simulink model "fi_sc"  (R2026a)
settings: Solver=VariableStepAuto  StopTime=40  FixedStep=0.1  MaxStep=.1
model workspace (MAT data in the model file):
  T = [0 0.05 0.1 0.15 0.2 0.25 0.3 0.35 0.4 0.45 0.5 0.55 ... (701 elements, 701x1)]
  U = [3.99594136536 3.99594136536 3.99594136536 3.99594136536 3.99594136536 3.99594136536 3.99594136536 3.99594136536 3.99594136536 3.99594136536 3.99594136536 3.99594136536 ... (701 elements, 701x1)]
libraries: neural x11, simulink_extras x2
settings Model: Creator=syaghoub  LastModifiedBy=harry_31916
settings DataIOCC: ExternalInput=simin

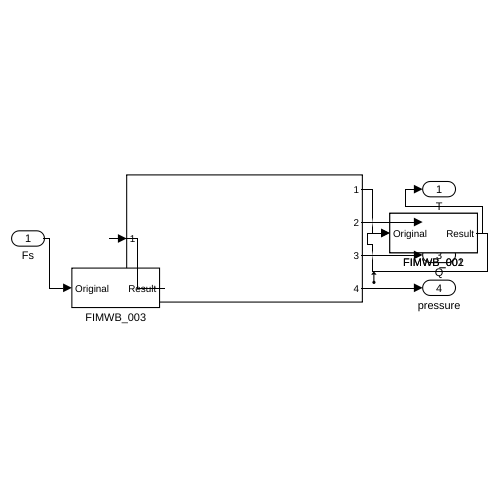
[thumbnail: Simulink's stored preview of the top-level diagram]
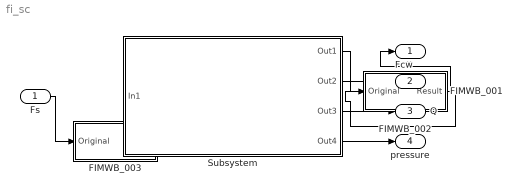
== system fi_sc ==
  Fs : Inport
  FIMWB_001 : Subsystem  Tag=fimwb.fault.1
  FIMWB_002 : Subsystem  Tag=fimwb.fault.2
  FIMWB_003 : Subsystem  Tag=fimwb.fault.3
  Subsystem : Subsystem
  T : Outport  VectorParamsAs1DForOutWhenUnconnected=off
  Fcw : Outport  Port=2  VectorParamsAs1DForOutWhenUnconnected=off
  Q : Outport  Port=3  VectorParamsAs1DForOutWhenUnconnected=off
  pressure : Outport  Port=4  VectorParamsAs1DForOutWhenUnconnected=off
  wires:
  Subsystem/2(Out2) -> Fcw/1
  Subsystem/3(Out3) -> Q/1
  Subsystem/4(Out4) -> pressure/1
  Subsystem/1(Out1) -> FIMWB_001/1(Original)
  FIMWB_001/1(Result) -> FIMWB_002/1(Original)
  FIMWB_002/1(Result) -> T/1
  Fs/1 -> FIMWB_003/1(Original)
  FIMWB_003/1(Result) -> Subsystem/1(In1)

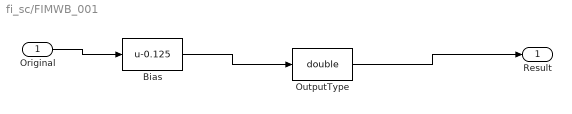
== system fi_sc/FIMWB_001 ==
  Original : Inport
  Bias : Bias  Bias=-0.125  SaturateOnIntegerOverflow=off
  OutputType : DataTypeConversion  OutDataTypeStr=double  RndMeth=Round
  Result : Outport
  wires:
  Original/1 -> Bias/1
  Bias/1 -> OutputType/1
  OutputType/1 -> Result/1

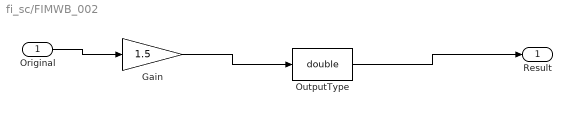
== system fi_sc/FIMWB_002 ==
  Original : Inport
  Gain : Gain  Gain=1.5  OutDataTypeStr=Inherit: Same as input
  OutputType : DataTypeConversion  OutDataTypeStr=double  RndMeth=Round
  Result : Outport
  wires:
  Original/1 -> Gain/1
  Gain/1 -> OutputType/1
  OutputType/1 -> Result/1

== system fi_sc/FIMWB_003 ==
  Original : Inport
  Bias : Bias  Bias=0.015625  SaturateOnIntegerOverflow=off
  OutputType : DataTypeConversion  OutDataTypeStr=double  RndMeth=Round
  Result : Outport
  wires:
  Original/1 -> Bias/1
  Bias/1 -> OutputType/1
  OutputType/1 -> Result/1

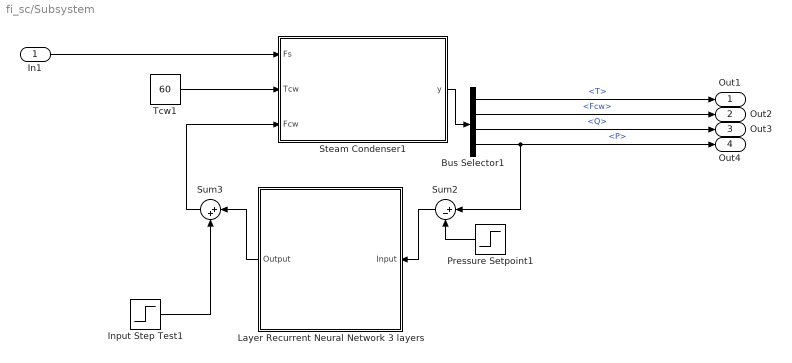
== system fi_sc/Subsystem ==
  In1 : Inport
  Bus Selector1 : BusSelector  OutputSignals=T,Fcw,Q,P
  Input Step Test1 : Step  Time=10  FinalValue=0  SampleTime=0
  "Layer Recurrent Neural Network 3 layers " : Subsystem  mask{ai_layer_1_delayed_1=[0;0;0], ai_layer_1_delayed_2=[0;0;0], Parameter3=[]}
      mask prompts: ai_layer_1_delayed_1 "Initial layer 1 state at timestep 0."; ai_layer_1_delayed_2 "Initial layer 1 state at timestep -1."
      mask help: Layer Recurrent Neural Network
      mask Display: e = 0.06;c1 = [120 150 230]/255;c2 = ([120 150 230]+0)/383;c3 = ([120 150 230]+128)/383;patch([0 1 1 0],[0 0 1 1],c1);patch([0 1 1 1-e 1-e 0+e],[0 0 1 1-e 0+e 0+e],c2);patch([0 0 1 1-e 0+e 0+e],[0 1 1 1-e 1-e 0+e],c3);plot([0 1 1 0 0],[0 0 1 1 0]);fprintf('NNET');port_label('input',1,' Input');port_label('output',1,'Output ');
  Pressure Setpoint1 : Step  Time=2  InitialValue=90  FinalValue=87  SampleTime=0
  Steam Condenser1 : Subsystem  mask{V=3, Mcw=500, UA=356.972413581334, tau=1, Fcw=107.8880952381, P=90, T=80}
      mask prompts: V "Volume [m3]"; Mcw "CW Holdup [kg]"; UA "UA [kW/K]"; tau "Actuator time constant [s]"; Fcw "Fcw [kg/s]"; P "P [kPa]"; T "T [degC]"
      mask init:
      | y1=[.3 .3 .7 .7 .3 NaN .4 .4 NaN .5 .5 NaN .6 .6 NaN 0.2 0.3 NaN 0.7 0.8 NaN 0.7 0.8 NaN 0.82 NaN 0.18];
      | x1=[.8 .2 .2 .8 .8 NaN .8 .2 NaN .8 .2 NaN .8 .2 NaN 0.5 0.5 NaN 0.3 0.3 NaN 0.7 0.7 NaN -0.05 NaN 1.05];
      | y2=0.3:0.05:0.7;
      | x2=sqrt(0.0625-(y2-0.5).^2);
      | y3=[.5 .5 .8 NaN 0.2 0.4 0.4];
      | x3=[x2(5)+0.65 0.95 0.95 NaN .1 .1 0.35-x2(3)];
      mask Display:
      | plot([x1 NaN 0.65+x2 NaN 0.35-x2 NaN x3],[y1 NaN y2 NaN y2 NaN y3])
      | port_label('input',1,'Fs')
      | port_label('input',2,'Tcw')
      | port_label('input',3,'Fcw')
      | port_label('output',1,'y')
  Sum2 : Sum  Inputs=|+-  InputSameDT=on  OutDataTypeStr=Inherit: Same as first input
  Sum3 : Sum  Inputs=|++  InputSameDT=on  OutDataTypeStr=Inherit: Same as first input
  Tcw1 : Constant  Value=60  VectorParams1D=off
  Out1 : Outport  VectorParamsAs1DForOutWhenUnconnected=off
  Out2 : Outport  Port=2  VectorParamsAs1DForOutWhenUnconnected=off
  Out3 : Outport  Port=3  VectorParamsAs1DForOutWhenUnconnected=off
  Out4 : Outport  Port=4  VectorParamsAs1DForOutWhenUnconnected=off
  wires:
  Bus Selector1/4 -> Out4/1, Sum2/1  "<P>"
  Bus Selector1/3 -> Out3/1  "<Q>"
  Tcw1/1 -> Steam Condenser1/2(Tcw)
  Sum3/1 -> Steam Condenser1/3(Fcw)
  Bus Selector1/1 -> Out1/1  "<T>"
  Steam Condenser1/1(y) -> Bus Selector1/1
  Bus Selector1/2 -> Out2/1  "<Fcw>"
  Pressure Setpoint1/1 -> Sum2/2
  Input Step Test1/1 -> Sum3/2
  In1/1 -> Steam Condenser1/1(Fs)
  Sum2/1 -> "Layer Recurrent Neural Network 3 layers "/1(Input)
  "Layer Recurrent Neural Network 3 layers "/1(Output) -> Sum3/1

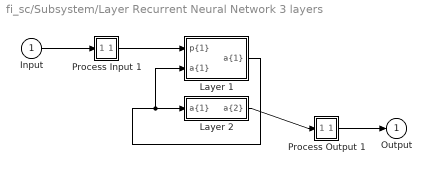
== system fi_sc/Subsystem/Layer Recurrent Neural Network 3 layers  ==
  Input : Inport  PortDimensions=1
      mask Display: e = 0.06;c1 = [120 230 180]/255;c2 = ([120 230 180]+0)/(256+128);c3 = ([120 230 180]+128)/(256+128);patch([0 1 1 0],[0 0 1 1],c1);patch([0 1 1 1-e 1-e 0+e],[0 0 1 1-e 0+e 0+e],c2);patch([0 0 1 1-e 0+e 0+e],[0 1 1 1-e 1-e 0+e],c3);plot([0 1 1 0 0],[0 0 1 1 0]);
  Layer 1 : Subsystem
      mask Display: e = 0.06;c1 = [120 150 230]/255;c2 = ([120 150 230]+0)/383;c3 = ([120 150 230]+128)/383;patch([0 1 1 0],[0 0 1 1],c1);patch([0 1 1 1-e 1-e 0+e],[0 0 1 1-e 0+e 0+e],c2);patch([0 0 1 1-e 0+e 0+e],[0 1 1 1-e 1-e 0+e],c3);plot([0 1 1 0 0],[0 0 1 1 0]);
  Layer 2 : Subsystem
      mask Display: e = 0.06;c1 = [120 150 230]/255;c2 = ([120 150 230]+0)/383;c3 = ([120 150 230]+128)/383;patch([0 1 1 0],[0 0 1 1],c1);patch([0 1 1 1-e 1-e 0+e],[0 0 1 1-e 0+e 0+e],c2);patch([0 0 1 1-e 0+e 0+e],[0 1 1 1-e 1-e 0+e],c3);plot([0 1 1 0 0],[0 0 1 1 0]);
  Process Input 1 : Subsystem
      mask Display: e = 0.06;c1 = [120 150 230]/255;c2 = ([120 150 230]+0)/383;c3 = ([120 150 230]+128)/383;patch([0 1 1 0],[0 0 1 1],c1);patch([0 1 1 1-e 1-e 0+e],[0 0 1 1-e 0+e 0+e],c2);patch([0 0 1 1-e 0+e 0+e],[0 1 1 1-e 1-e 0+e],c3);plot([0 1 1 0 0],[0 0 1 1 0]);
  Process Output 1 : Subsystem
      mask Display: e = 0.06;c1 = [120 150 230]/255;c2 = ([120 150 230]+0)/383;c3 = ([120 150 230]+128)/383;patch([0 1 1 0],[0 0 1 1],c1);patch([0 1 1 1-e 1-e 0+e],[0 0 1 1-e 0+e 0+e],c2);patch([0 0 1 1-e 0+e 0+e],[0 1 1 1-e 1-e 0+e],c3);plot([0 1 1 0 0],[0 0 1 1 0]);
  Output : Outport  InitialOutput=0  VectorParamsAs1DForOutWhenUnconnected=off
      mask Display: e = 0.06;c1 = [120 230 180]/255;c2 = ([120 230 180]+0)/(256+128);c3 = ([120 230 180]+128)/(256+128);patch([0 1 1 0],[0 0 1 1],c1);patch([0 1 1 1-e 1-e 0+e],[0 0 1 1-e 0+e 0+e],c2);patch([0 0 1 1-e 0+e 0+e],[0 1 1 1-e 1-e 0+e],c3);plot([0 1 1 0 0],[0 0 1 1 0]);
  wires:
  Layer 1/1("a{1}") -> Layer 1/2("a{1} "), Layer 2/1("a{1} ")
  Process Input 1/1(p) -> Layer 1/1("p{1}")
  Layer 2/1("a{2}") -> Process Output 1/1(a)
  Input/1 -> Process Input 1/1(x)
  Process Output 1/1(y) -> Output/1

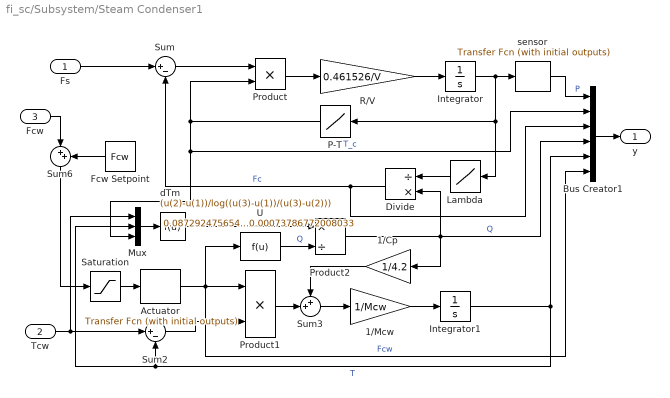
== system fi_sc/Subsystem/Steam Condenser1 ==
  Fs : Inport
  Tcw : Inport  Port=2
  Fcw : Inport  Port=3
  1/Cp : Gain  Gain=1/4.2  OutDataTypeStr=Inherit: Same as input  ParamDataTypeStr=Inherit: Same as input
  1/Mcw : Gain  Gain=1/Mcw  OutDataTypeStr=Inherit: Same as input  ParamDataTypeStr=Inherit: Same as input
  Actuator : simulink_extras/Additional Linear/Transfer Fcn (with initial outputs)  N=[1]  D=[tau 1]  Y0=Fcw  U0=Fcw
  Bus Creator1 : BusCreator  Inputs=6
  Divide : Product  Inputs=/*  InputSameDT=on  RndMeth=Zero  OutDataTypeStr=Inherit: Same as first input
  Fcw Setpoint : Constant  Value=Fcw
  Integrator : Integrator  InitialCondition=P
  Integrator1 : Integrator  InitialCondition=T
  Lambda : Lookup  InputValues=[50 60 70 80 90 100 110]  Table=[2305.42 2293.64 2283.30 2274.05 2265.65 2257.92 2250.76]
  Mux : Mux  Inputs=3
  P-T : Lookup  InputValues=[50 60 70 80 90 100 110]  Table=[81.3167 85.9258 89.9315 93.4854 96.6870 99.6059 102.2923]
  Product : Product  InputSameDT=on  RndMeth=Zero  OutDataTypeStr=Inherit: Same as first input
  Product1 : Product  InputSameDT=on  RndMeth=Zero  OutDataTypeStr=Inherit: Same as first input
  Product2 : Product  Inputs=*/  InputSameDT=on  RndMeth=Zero  OutDataTypeStr=Inherit: Same as first input
  R/V : Gain  Gain=0.461526/V  OutDataTypeStr=Inherit: Same as input  ParamDataTypeStr=Inherit: Same as input
  Saturation : Saturate  UpperLimit=200  LowerLimit=0
  Sum : Sum  Inputs=|+-  InputSameDT=on  OutDataTypeStr=Inherit: Same as first input
  Sum2 : Sum  Inputs=|+-  InputSameDT=on  OutDataTypeStr=Inherit: Same as first input
  Sum3 : Sum  Inputs=++|  InputSameDT=on  OutDataTypeStr=Inherit: Same as first input
  Sum6 : Sum  Inputs=|++  InputSameDT=on  OutDataTypeStr=Inherit: Same as first input
  U : Fcn  Expr=0.0872924756541668/u^0.8+0.00073786772008033
  dTm : Fcn  Expr=(u(2)-u(1))/log((u(3)-u(1))/(u(3)-u(2)))
  sensor : simulink_extras/Additional Linear/Transfer Fcn (with initial outputs)  N=[1]  D=[tau/2 1]  Y0=P  U0=P
  y : Outport  VectorParamsAs1DForOutWhenUnconnected=off
  wires:
  R/V/1 -> Integrator/1
  Product/1 -> R/V/1
  Sum/1 -> Product/1
  Fs/1 -> Sum/1
  Integrator/1 -> sensor/1, Lambda/1, P-T/1
  1/Mcw/1 -> Integrator1/1
  Integrator1/1 -> Sum2/2, Mux/2, Bus Creator1/5  "T"
  Tcw/1 -> Sum2/1, Mux/1
  Sum2/1 -> Product1/2
  Product1/1 -> Sum3/2
  Sum3/1 -> 1/Mcw/1
  1/Cp/1 -> Sum3/1
  dTm/1 -> Product2/1
  Bus Creator1/1 -> y/1
  Actuator/1 -> Product1/1, U/1, Bus Creator1/6  "Fcw"
  sensor/1 -> Bus Creator1/1  "P"
  Saturation/1 -> Actuator/1
  Sum6/1 -> Saturation/1
  Fcw/1 -> Sum6/1
  Fcw Setpoint/1 -> Sum6/2
  Lambda/1 -> Divide/1
  Divide/1 -> Sum/2, Bus Creator1/3  "Fc"
  P-T/1 -> Product/2, Mux/3, Bus Creator1/2  "T_c"
  Mux/1 -> dTm/1
  Product2/1 -> 1/Cp/1, Divide/2, Bus Creator1/4  "Q"
  U/1 -> Product2/2  "Q"

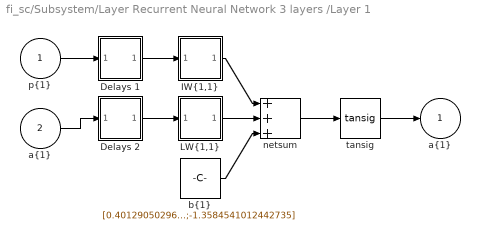
== system fi_sc/Subsystem/Layer Recurrent Neural Network 3 layers /Layer 1 ==
  "p{1}" : Inport  PortDimensions=1
      mask Display: e = 0.06;c1 = [120 230 180]/255;c2 = ([120 230 180]+0)/(256+128);c3 = ([120 230 180]+128)/(256+128);patch([0 1 1 0],[0 0 1 1],c1);patch([0 1 1 1-e 1-e 0+e],[0 0 1 1-e 0+e 0+e],c2);patch([0 0 1 1-e 0+e 0+e],[0 1 1 1-e 1-e 0+e],c3);plot([0 1 1 0 0],[0 0 1 1 0]);
  "a{1} " : Inport  Port=2  PortDimensions=3
      mask Display: e = 0.06;c1 = [120 230 180]/255;c2 = ([120 230 180]+0)/(256+128);c3 = ([120 230 180]+128)/(256+128);patch([0 1 1 0],[0 0 1 1],c1);patch([0 1 1 1-e 1-e 0+e],[0 0 1 1-e 0+e 0+e],c2);patch([0 0 1 1-e 0+e 0+e],[0 1 1 1-e 1-e 0+e],c3);plot([0 1 1 0 0],[0 0 1 1 0]);
  Delays 1 : Subsystem
      mask Display: e = 0.06;c1 = [120 150 230]/255;c2 = ([120 150 230]+0)/383;c3 = ([120 150 230]+128)/383;patch([0 1 1 0],[0 0 1 1],c1);patch([0 1 1 1-e 1-e 0+e],[0 0 1 1-e 0+e 0+e],c2);patch([0 0 1 1-e 0+e 0+e],[0 1 1 1-e 1-e 0+e],c3);plot([0 1 1 0 0],[0 0 1 1 0]);disp('0');
  Delays 2 : Subsystem
      mask Display: e = 0.06;c1 = [120 150 230]/255;c2 = ([120 150 230]+0)/383;c3 = ([120 150 230]+128)/383;patch([0 1 1 0],[0 0 1 1],c1);patch([0 1 1 1-e 1-e 0+e],[0 0 1 1-e 0+e 0+e],c2);patch([0 0 1 1-e 0+e 0+e],[0 1 1 1-e 1-e 0+e],c3);plot([0 1 1 0 0],[0 0 1 1 0]);disp('1-2');
  "IW{1,1}" : Subsystem
      mask Display: e = 0.06;c1 = [120 150 230]/255;c2 = ([120 150 230]+0)/383;c3 = ([120 150 230]+128)/383;patch([0 1 1 0],[0 0 1 1],c1);patch([0 1 1 1-e 1-e 0+e],[0 0 1 1-e 0+e 0+e],c2);patch([0 0 1 1-e 0+e 0+e],[0 1 1 1-e 1-e 0+e],c3);plot([0 1 1 0 0],[0 0 1 1 0]);disp('W');
  "LW{1,1}" : Subsystem
      mask Display: e = 0.06;c1 = [120 150 230]/255;c2 = ([120 150 230]+0)/383;c3 = ([120 150 230]+128)/383;patch([0 1 1 0],[0 0 1 1],c1);patch([0 1 1 1-e 1-e 0+e],[0 0 1 1-e 0+e 0+e],c2);patch([0 0 1 1-e 0+e 0+e],[0 1 1 1-e 1-e 0+e],c3);plot([0 1 1 0 0],[0 0 1 1 0]);disp('W');
  "b{1}" : Constant  Value=[0.40129050296348601;-0.12475735064274925;-1.3584541012442735]
      mask Display: e = 0.06;c1 = [120 150 230]/255;c2 = ([120 150 230]+0)/383;c3 = ([120 150 230]+128)/383;patch([0 1 1 0],[0 0 1 1],c1);patch([0 1 1 1-e 1-e 0+e],[0 0 1 1-e 0+e 0+e],c2);patch([0 0 1 1-e 0+e 0+e],[0 1 1 1-e 1-e 0+e],c3);plot([0 1 1 0 0],[0 0 1 1 0]);disp('b');
  netsum : Sum  Inputs=3  InputSameDT=on  SaturateOnIntegerOverflow=on  OutDataTypeStr=Inherit: Same as first input
      mask Display: e = 0.06;c1 = [120 150 230]/255;c2 = ([120 150 230]+0)/383;c3 = ([120 150 230]+128)/383;patch([0 1 1 0],[0 0 1 1],c1);patch([0 1 1 1-e 1-e 0+e],[0 0 1 1-e 0+e 0+e],c2);patch([0 0 1 1-e 0+e 0+e],[0 1 1 1-e 1-e 0+e],c3);plot([0 1 1 0 0],[0 0 1 1 0]);disp('+');
  tansig : neural/Transfer Functions/tansig
  "a{1}" : Outport  InitialOutput=[0;0;0]  VectorParamsAs1DForOutWhenUnconnected=off
      mask Display: e = 0.06;c1 = [120 230 180]/255;c2 = ([120 230 180]+0)/(256+128);c3 = ([120 230 180]+128)/(256+128);patch([0 1 1 0],[0 0 1 1],c1);patch([0 1 1 1-e 1-e 0+e],[0 0 1 1-e 0+e 0+e],c2);patch([0 0 1 1-e 0+e 0+e],[0 1 1 1-e 1-e 0+e],c3);plot([0 1 1 0 0],[0 0 1 1 0]);
  wires:
  "p{1}"/1 -> Delays 1/1("p{1}")
  Delays 1/1("pd{1,1}") -> "IW{1,1}"/1("pd{1,1}")
  "IW{1,1}"/1("iz{1,1}") -> netsum/1
  "a{1} "/1 -> Delays 2/1("p{1}")
  Delays 2/1("pd{1,1}") -> "LW{1,1}"/1("ad{1,1}")
  "LW{1,1}"/1("lz{1,1}") -> netsum/2
  "b{1}"/1 -> netsum/3
  netsum/1 -> tansig/1
  tansig/1 -> "a{1}"/1

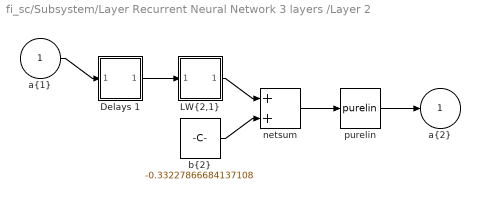
== system fi_sc/Subsystem/Layer Recurrent Neural Network 3 layers /Layer 2 ==
  "a{1} " : Inport  PortDimensions=3
      mask Display: e = 0.06;c1 = [120 230 180]/255;c2 = ([120 230 180]+0)/(256+128);c3 = ([120 230 180]+128)/(256+128);patch([0 1 1 0],[0 0 1 1],c1);patch([0 1 1 1-e 1-e 0+e],[0 0 1 1-e 0+e 0+e],c2);patch([0 0 1 1-e 0+e 0+e],[0 1 1 1-e 1-e 0+e],c3);plot([0 1 1 0 0],[0 0 1 1 0]);
  Delays 1 : Subsystem
      mask Display: e = 0.06;c1 = [120 150 230]/255;c2 = ([120 150 230]+0)/383;c3 = ([120 150 230]+128)/383;patch([0 1 1 0],[0 0 1 1],c1);patch([0 1 1 1-e 1-e 0+e],[0 0 1 1-e 0+e 0+e],c2);patch([0 0 1 1-e 0+e 0+e],[0 1 1 1-e 1-e 0+e],c3);plot([0 1 1 0 0],[0 0 1 1 0]);disp('0');
  "LW{2,1}" : Subsystem
      mask Display: e = 0.06;c1 = [120 150 230]/255;c2 = ([120 150 230]+0)/383;c3 = ([120 150 230]+128)/383;patch([0 1 1 0],[0 0 1 1],c1);patch([0 1 1 1-e 1-e 0+e],[0 0 1 1-e 0+e 0+e],c2);patch([0 0 1 1-e 0+e 0+e],[0 1 1 1-e 1-e 0+e],c3);plot([0 1 1 0 0],[0 0 1 1 0]);disp('W');
  "b{2}" : Constant  Value=-0.33227866684137108
      mask Display: e = 0.06;c1 = [120 150 230]/255;c2 = ([120 150 230]+0)/383;c3 = ([120 150 230]+128)/383;patch([0 1 1 0],[0 0 1 1],c1);patch([0 1 1 1-e 1-e 0+e],[0 0 1 1-e 0+e 0+e],c2);patch([0 0 1 1-e 0+e 0+e],[0 1 1 1-e 1-e 0+e],c3);plot([0 1 1 0 0],[0 0 1 1 0]);disp('b');
  netsum : Sum  Inputs=2  InputSameDT=on  SaturateOnIntegerOverflow=on  OutDataTypeStr=Inherit: Same as first input
      mask Display: e = 0.06;c1 = [120 150 230]/255;c2 = ([120 150 230]+0)/383;c3 = ([120 150 230]+128)/383;patch([0 1 1 0],[0 0 1 1],c1);patch([0 1 1 1-e 1-e 0+e],[0 0 1 1-e 0+e 0+e],c2);patch([0 0 1 1-e 0+e 0+e],[0 1 1 1-e 1-e 0+e],c3);plot([0 1 1 0 0],[0 0 1 1 0]);disp('+');
  purelin : neural/Transfer Functions/purelin
  "a{2}" : Outport  InitialOutput=0  VectorParamsAs1DForOutWhenUnconnected=off
      mask Display: e = 0.06;c1 = [120 230 180]/255;c2 = ([120 230 180]+0)/(256+128);c3 = ([120 230 180]+128)/(256+128);patch([0 1 1 0],[0 0 1 1],c1);patch([0 1 1 1-e 1-e 0+e],[0 0 1 1-e 0+e 0+e],c2);patch([0 0 1 1-e 0+e 0+e],[0 1 1 1-e 1-e 0+e],c3);plot([0 1 1 0 0],[0 0 1 1 0]);
  wires:
  "a{1} "/1 -> Delays 1/1("p{2}")
  Delays 1/1("pd{2,1}") -> "LW{2,1}"/1("ad{2,1}")
  "LW{2,1}"/1("lz{2,1}") -> netsum/1
  "b{2}"/1 -> netsum/2
  netsum/1 -> purelin/1
  purelin/1 -> "a{2}"/1

== system fi_sc/Subsystem/Layer Recurrent Neural Network 3 layers /Process Input 1 ==
  x : Inport  PortDimensions=1
      mask Display: e = 0.06;c1 = [120 230 180]/255;c2 = ([120 230 180]+0)/(256+128);c3 = ([120 230 180]+128)/(256+128);patch([0 1 1 0],[0 0 1 1],c1);patch([0 1 1 1-e 1-e 0+e],[0 0 1 1-e 0+e 0+e],c2);patch([0 0 1 1-e 0+e 0+e],[0 1 1 1-e 1-e 0+e],c3);plot([0 1 1 0 0],[0 0 1 1 0]);
  mapminmax : neural/Processing Functions/mapminmax  xmin=-3.7742393716738434  xmax=5.7997431225043385  ymin=-1  ymax=1
  p : Outport  PortDimensions=1  VectorParamsAs1DForOutWhenUnconnected=off
      mask Display: e = 0.06;c1 = [120 230 180]/255;c2 = ([120 230 180]+0)/(256+128);c3 = ([120 230 180]+128)/(256+128);patch([0 1 1 0],[0 0 1 1],c1);patch([0 1 1 1-e 1-e 0+e],[0 0 1 1-e 0+e 0+e],c2);patch([0 0 1 1-e 0+e 0+e],[0 1 1 1-e 1-e 0+e],c3);plot([0 1 1 0 0],[0 0 1 1 0]);
  wires:
  x/1 -> mapminmax/1
  mapminmax/1 -> p/1

== system fi_sc/Subsystem/Layer Recurrent Neural Network 3 layers /Process Output 1 ==
  a : Inport  PortDimensions=1
      mask Display: e = 0.06;c1 = [120 230 180]/255;c2 = ([120 230 180]+0)/(256+128);c3 = ([120 230 180]+128)/(256+128);patch([0 1 1 0],[0 0 1 1],c1);patch([0 1 1 1-e 1-e 0+e],[0 0 1 1-e 0+e 0+e],c2);patch([0 0 1 1-e 0+e 0+e],[0 1 1 1-e 1-e 0+e],c3);plot([0 1 1 0 0],[0 0 1 1 0]);
  mapminmax_reverse : neural/Processing Functions/mapminmax_reverse  xmin=-30.855068745036114  xmax=66.879264965962932  ymin=-1  ymax=1
  y : Outport  PortDimensions=1  VectorParamsAs1DForOutWhenUnconnected=off
      mask Display: e = 0.06;c1 = [120 230 180]/255;c2 = ([120 230 180]+0)/(256+128);c3 = ([120 230 180]+128)/(256+128);patch([0 1 1 0],[0 0 1 1],c1);patch([0 1 1 1-e 1-e 0+e],[0 0 1 1-e 0+e 0+e],c2);patch([0 0 1 1-e 0+e 0+e],[0 1 1 1-e 1-e 0+e],c3);plot([0 1 1 0 0],[0 0 1 1 0]);
  wires:
  a/1 -> mapminmax_reverse/1
  mapminmax_reverse/1 -> y/1

== system fi_sc/Subsystem/Layer Recurrent Neural Network 3 layers /Layer 1/Delays 1 ==
  "p{1}" : Inport  PortDimensions=1
      mask Display: e = 0.06;c1 = [120 230 180]/255;c2 = ([120 230 180]+0)/(256+128);c3 = ([120 230 180]+128)/(256+128);patch([0 1 1 0],[0 0 1 1],c1);patch([0 1 1 1-e 1-e 0+e],[0 0 1 1-e 0+e 0+e],c2);patch([0 0 1 1-e 0+e 0+e],[0 1 1 1-e 1-e 0+e],c3);plot([0 1 1 0 0],[0 0 1 1 0]);
  mux : Mux  Inputs=1
      mask Display: e = 0.06;c1 = [120 150 230]/255;c2 = ([120 150 230]+0)/383;c3 = ([120 150 230]+128)/383;patch([0 1 1 0],[0 0 1 1],c1);patch([0 1 1 1-e 1-e 0+e],[0 0 1 1-e 0+e 0+e],c2);patch([0 0 1 1-e 0+e 0+e],[0 1 1 1-e 1-e 0+e],c3);plot([0 1 1 0 0],[0 0 1 1 0]);disp('Mux')
  "pd{1,1}" : Outport  VectorParamsAs1DForOutWhenUnconnected=off
      mask Display: e = 0.06;c1 = [120 230 180]/255;c2 = ([120 230 180]+0)/(256+128);c3 = ([120 230 180]+128)/(256+128);patch([0 1 1 0],[0 0 1 1],c1);patch([0 1 1 1-e 1-e 0+e],[0 0 1 1-e 0+e 0+e],c2);patch([0 0 1 1-e 0+e 0+e],[0 1 1 1-e 1-e 0+e],c3);plot([0 1 1 0 0],[0 0 1 1 0]);
  wires:
  "p{1}"/1 -> mux/1
  mux/1 -> "pd{1,1}"/1

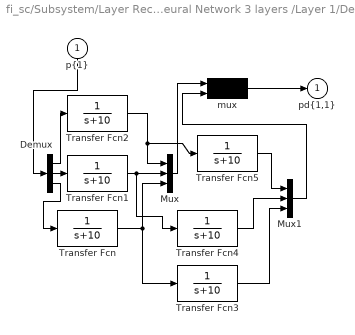
== system fi_sc/Subsystem/Layer Recurrent Neural Network 3 layers /Layer 1/Delays 2 ==
  "p{1}" : Inport  PortDimensions=3
      mask Display: e = 0.06;c1 = [120 230 180]/255;c2 = ([120 230 180]+0)/(256+128);c3 = ([120 230 180]+128)/(256+128);patch([0 1 1 0],[0 0 1 1],c1);patch([0 1 1 1-e 1-e 0+e],[0 0 1 1-e 0+e 0+e],c2);patch([0 0 1 1-e 0+e 0+e],[0 1 1 1-e 1-e 0+e],c3);plot([0 1 1 0 0],[0 0 1 1 0]);
  Demux : Demux  Outputs=3
  Mux : Mux  Inputs=3
  Mux1 : Mux  Inputs=3
  Transfer Fcn{,1..5} (6 alike) : TransferFcn  Denominator=[1 10]
  mux : Mux  Inputs=2
      mask Display: e = 0.06;c1 = [120 150 230]/255;c2 = ([120 150 230]+0)/383;c3 = ([120 150 230]+128)/383;patch([0 1 1 0],[0 0 1 1],c1);patch([0 1 1 1-e 1-e 0+e],[0 0 1 1-e 0+e 0+e],c2);patch([0 0 1 1-e 0+e 0+e],[0 1 1 1-e 1-e 0+e],c3);plot([0 1 1 0 0],[0 0 1 1 0]);disp('Mux')
  "pd{1,1}" : Outport  VectorParamsAs1DForOutWhenUnconnected=off
      mask Display: e = 0.06;c1 = [120 230 180]/255;c2 = ([120 230 180]+0)/(256+128);c3 = ([120 230 180]+128)/(256+128);patch([0 1 1 0],[0 0 1 1],c1);patch([0 1 1 1-e 1-e 0+e],[0 0 1 1-e 0+e 0+e],c2);patch([0 0 1 1-e 0+e 0+e],[0 1 1 1-e 1-e 0+e],c3);plot([0 1 1 0 0],[0 0 1 1 0]);
  wires:
  "p{1}"/1 -> Demux/1
  mux/1 -> "pd{1,1}"/1
  Transfer Fcn/1 -> Transfer Fcn3/1, Mux/3
  Demux/3 -> Transfer Fcn/1
  Demux/1 -> Transfer Fcn2/1
  Demux/2 -> Transfer Fcn1/1
  Mux1/1 -> mux/2
  Transfer Fcn2/1 -> Transfer Fcn5/1, Mux/1
  Transfer Fcn1/1 -> Transfer Fcn4/1, Mux/2
  Mux/1 -> mux/1
  Transfer Fcn3/1 -> Mux1/3
  Transfer Fcn4/1 -> Mux1/2
  Transfer Fcn5/1 -> Mux1/1

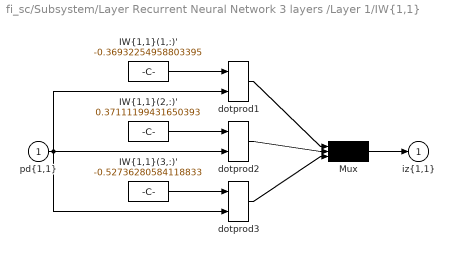
== system fi_sc/Subsystem/Layer Recurrent Neural Network 3 layers /Layer 1/IW{1,1} ==
  "pd{1,1}" : Inport  PortDimensions=1
      mask Display: e = 0.06;c1 = [120 230 180]/255;c2 = ([120 230 180]+0)/(256+128);c3 = ([120 230 180]+128)/(256+128);patch([0 1 1 0],[0 0 1 1],c1);patch([0 1 1 1-e 1-e 0+e],[0 0 1 1-e 0+e 0+e],c2);patch([0 0 1 1-e 0+e 0+e],[0 1 1 1-e 1-e 0+e],c3);plot([0 1 1 0 0],[0 0 1 1 0]);
  "IW{1,1}(1,:)'" : Constant  Value=-0.36932254958803395
      mask Display: e = 0.06;c1 = [120 150 230]/255;c2 = ([120 150 230]+0)/383;c3 = ([120 150 230]+128)/383;patch([0 1 1 0],[0 0 1 1],c1);patch([0 1 1 1-e 1-e 0+e],[0 0 1 1-e 0+e 0+e],c2);patch([0 0 1 1-e 0+e 0+e],[0 1 1 1-e 1-e 0+e],c3);plot([0 1 1 0 0],[0 0 1 1 0]);disp('Weights');
  "IW{1,1}(2,:)'" : Constant  Value=0.37111199431650393
      mask Display: e = 0.06;c1 = [120 150 230]/255;c2 = ([120 150 230]+0)/383;c3 = ([120 150 230]+128)/383;patch([0 1 1 0],[0 0 1 1],c1);patch([0 1 1 1-e 1-e 0+e],[0 0 1 1-e 0+e 0+e],c2);patch([0 0 1 1-e 0+e 0+e],[0 1 1 1-e 1-e 0+e],c3);plot([0 1 1 0 0],[0 0 1 1 0]);disp('Weights');
  "IW{1,1}(3,:)'" : Constant  Value=-0.52736280584118833
      mask Display: e = 0.06;c1 = [120 150 230]/255;c2 = ([120 150 230]+0)/383;c3 = ([120 150 230]+128)/383;patch([0 1 1 0],[0 0 1 1],c1);patch([0 1 1 1-e 1-e 0+e],[0 0 1 1-e 0+e 0+e],c2);patch([0 0 1 1-e 0+e 0+e],[0 1 1 1-e 1-e 0+e],c3);plot([0 1 1 0 0],[0 0 1 1 0]);disp('Weights');
  Mux : Mux  Inputs=3
      mask Display: e = 0.06;c1 = [120 150 230]/255;c2 = ([120 150 230]+0)/383;c3 = ([120 150 230]+128)/383;patch([0 1 1 0],[0 0 1 1],c1);patch([0 1 1 1-e 1-e 0+e],[0 0 1 1-e 0+e 0+e],c2);patch([0 0 1 1-e 0+e 0+e],[0 1 1 1-e 1-e 0+e],c3);plot([0 1 1 0 0],[0 0 1 1 0]);disp('Mux');
  dotprod1 : neural/Weight Functions/dotprod
  dotprod2 : neural/Weight Functions/dotprod
  dotprod3 : neural/Weight Functions/dotprod
  "iz{1,1}" : Outport  VectorParamsAs1DForOutWhenUnconnected=off
      mask Display: e = 0.06;c1 = [120 230 180]/255;c2 = ([120 230 180]+0)/(256+128);c3 = ([120 230 180]+128)/(256+128);patch([0 1 1 0],[0 0 1 1],c1);patch([0 1 1 1-e 1-e 0+e],[0 0 1 1-e 0+e 0+e],c2);patch([0 0 1 1-e 0+e 0+e],[0 1 1 1-e 1-e 0+e],c3);plot([0 1 1 0 0],[0 0 1 1 0]);
  wires:
  "IW{1,1}(1,:)'"/1 -> dotprod1/1
  "pd{1,1}"/1 -> dotprod1/2, dotprod2/2, dotprod3/2
  dotprod1/1 -> Mux/1
  "IW{1,1}(2,:)'"/1 -> dotprod2/1
  dotprod2/1 -> Mux/2
  "IW{1,1}(3,:)'"/1 -> dotprod3/1
  dotprod3/1 -> Mux/3
  Mux/1 -> "iz{1,1}"/1

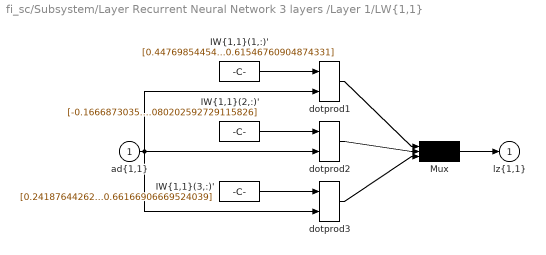
== system fi_sc/Subsystem/Layer Recurrent Neural Network 3 layers /Layer 1/LW{1,1} ==
  "ad{1,1}" : Inport  PortDimensions=6
      mask Display: e = 0.06;c1 = [120 230 180]/255;c2 = ([120 230 180]+0)/(256+128);c3 = ([120 230 180]+128)/(256+128);patch([0 1 1 0],[0 0 1 1],c1);patch([0 1 1 1-e 1-e 0+e],[0 0 1 1-e 0+e 0+e],c2);patch([0 0 1 1-e 0+e 0+e],[0 1 1 1-e 1-e 0+e],c3);plot([0 1 1 0 0],[0 0 1 1 0]);
  "IW{1,1}(1,:)'" : Constant  Value=[0.44769854454577174;1.1961840315574388;1.1412233787458486;0.72001623019786209;-0.37547125154051064;-0.61546760904874331]
      mask Display: e = 0.06;c1 = [120 150 230]/255;c2 = ([120 150 230]+0)/383;c3 = ([120 150 230]+128)/383;patch([0 1 1 0],[0 0 1 1],c1);patch([0 1 1 1-e 1-e 0+e],[0 0 1 1-e 0+e 0+e],c2);patch([0 0 1 1-e 0+e 0+e],[0 1 1 1-e 1-e 0+e],c3);plot([0 1 1 0 0],[0 0 1 1 0]);disp('weights');
  "IW{1,1}(2,:)'" : Constant  Value=[-0.16668730359454359;-0.016432941671533533;-0.22132796342367161;-0.037206224095552992;0.059874671921603305;0.080202592729115826]
      mask Display: e = 0.06;c1 = [120 150 230]/255;c2 = ([120 150 230]+0)/383;c3 = ([120 150 230]+128)/383;patch([0 1 1 0],[0 0 1 1],c1);patch([0 1 1 1-e 1-e 0+e],[0 0 1 1-e 0+e 0+e],c2);patch([0 0 1 1-e 0+e 0+e],[0 1 1 1-e 1-e 0+e],c3);plot([0 1 1 0 0],[0 0 1 1 0]);disp('weights');
  "IW{1,1}(3,:)'" : Constant  Value=[0.24187644262601646;-0.66963285238228187;-1.0984401489322673;0.029109804692608397;1.3722216833345802;0.66166906669524039]
      mask Display: e = 0.06;c1 = [120 150 230]/255;c2 = ([120 150 230]+0)/383;c3 = ([120 150 230]+128)/383;patch([0 1 1 0],[0 0 1 1],c1);patch([0 1 1 1-e 1-e 0+e],[0 0 1 1-e 0+e 0+e],c2);patch([0 0 1 1-e 0+e 0+e],[0 1 1 1-e 1-e 0+e],c3);plot([0 1 1 0 0],[0 0 1 1 0]);disp('weights');
  Mux : Mux  Inputs=3
      mask Display: e = 0.06;c1 = [120 150 230]/255;c2 = ([120 150 230]+0)/383;c3 = ([120 150 230]+128)/383;patch([0 1 1 0],[0 0 1 1],c1);patch([0 1 1 1-e 1-e 0+e],[0 0 1 1-e 0+e 0+e],c2);patch([0 0 1 1-e 0+e 0+e],[0 1 1 1-e 1-e 0+e],c3);plot([0 1 1 0 0],[0 0 1 1 0]);disp('Mux');
  dotprod1 : neural/Weight Functions/dotprod
  dotprod2 : neural/Weight Functions/dotprod
  dotprod3 : neural/Weight Functions/dotprod
  "lz{1,1}" : Outport  VectorParamsAs1DForOutWhenUnconnected=off
      mask Display: e = 0.06;c1 = [120 230 180]/255;c2 = ([120 230 180]+0)/(256+128);c3 = ([120 230 180]+128)/(256+128);patch([0 1 1 0],[0 0 1 1],c1);patch([0 1 1 1-e 1-e 0+e],[0 0 1 1-e 0+e 0+e],c2);patch([0 0 1 1-e 0+e 0+e],[0 1 1 1-e 1-e 0+e],c3);plot([0 1 1 0 0],[0 0 1 1 0]);
  wires:
  "IW{1,1}(1,:)'"/1 -> dotprod1/1
  "ad{1,1}"/1 -> dotprod1/2, dotprod2/2, dotprod3/2
  dotprod1/1 -> Mux/1
  "IW{1,1}(2,:)'"/1 -> dotprod2/1
  dotprod2/1 -> Mux/2
  "IW{1,1}(3,:)'"/1 -> dotprod3/1
  dotprod3/1 -> Mux/3
  Mux/1 -> "lz{1,1}"/1

== system fi_sc/Subsystem/Layer Recurrent Neural Network 3 layers /Layer 2/Delays 1 ==
  "p{2}" : Inport  PortDimensions=3
      mask Display: e = 0.06;c1 = [120 230 180]/255;c2 = ([120 230 180]+0)/(256+128);c3 = ([120 230 180]+128)/(256+128);patch([0 1 1 0],[0 0 1 1],c1);patch([0 1 1 1-e 1-e 0+e],[0 0 1 1-e 0+e 0+e],c2);patch([0 0 1 1-e 0+e 0+e],[0 1 1 1-e 1-e 0+e],c3);plot([0 1 1 0 0],[0 0 1 1 0]);
  mux : Mux  Inputs=1
      mask Display: e = 0.06;c1 = [120 150 230]/255;c2 = ([120 150 230]+0)/383;c3 = ([120 150 230]+128)/383;patch([0 1 1 0],[0 0 1 1],c1);patch([0 1 1 1-e 1-e 0+e],[0 0 1 1-e 0+e 0+e],c2);patch([0 0 1 1-e 0+e 0+e],[0 1 1 1-e 1-e 0+e],c3);plot([0 1 1 0 0],[0 0 1 1 0]);disp('Mux')
  "pd{2,1}" : Outport  VectorParamsAs1DForOutWhenUnconnected=off
      mask Display: e = 0.06;c1 = [120 230 180]/255;c2 = ([120 230 180]+0)/(256+128);c3 = ([120 230 180]+128)/(256+128);patch([0 1 1 0],[0 0 1 1],c1);patch([0 1 1 1-e 1-e 0+e],[0 0 1 1-e 0+e 0+e],c2);patch([0 0 1 1-e 0+e 0+e],[0 1 1 1-e 1-e 0+e],c3);plot([0 1 1 0 0],[0 0 1 1 0]);
  wires:
  "p{2}"/1 -> mux/1
  mux/1 -> "pd{2,1}"/1

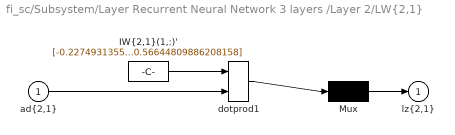
== system fi_sc/Subsystem/Layer Recurrent Neural Network 3 layers /Layer 2/LW{2,1} ==
  "ad{2,1}" : Inport  PortDimensions=3
      mask Display: e = 0.06;c1 = [120 230 180]/255;c2 = ([120 230 180]+0)/(256+128);c3 = ([120 230 180]+128)/(256+128);patch([0 1 1 0],[0 0 1 1],c1);patch([0 1 1 1-e 1-e 0+e],[0 0 1 1-e 0+e 0+e],c2);patch([0 0 1 1-e 0+e 0+e],[0 1 1 1-e 1-e 0+e],c3);plot([0 1 1 0 0],[0 0 1 1 0]);
  "IW{2,1}(1,:)'" : Constant  Value=[-0.22749313555095124;2.0804967759906643;-0.56644809886208158]
      mask Display: e = 0.06;c1 = [120 150 230]/255;c2 = ([120 150 230]+0)/383;c3 = ([120 150 230]+128)/383;patch([0 1 1 0],[0 0 1 1],c1);patch([0 1 1 1-e 1-e 0+e],[0 0 1 1-e 0+e 0+e],c2);patch([0 0 1 1-e 0+e 0+e],[0 1 1 1-e 1-e 0+e],c3);plot([0 1 1 0 0],[0 0 1 1 0]);disp('weights');
  Mux : Mux  Inputs=1
      mask Display: e = 0.06;c1 = [120 150 230]/255;c2 = ([120 150 230]+0)/383;c3 = ([120 150 230]+128)/383;patch([0 1 1 0],[0 0 1 1],c1);patch([0 1 1 1-e 1-e 0+e],[0 0 1 1-e 0+e 0+e],c2);patch([0 0 1 1-e 0+e 0+e],[0 1 1 1-e 1-e 0+e],c3);plot([0 1 1 0 0],[0 0 1 1 0]);disp('Mux');
  dotprod1 : neural/Weight Functions/dotprod
  "lz{2,1}" : Outport  VectorParamsAs1DForOutWhenUnconnected=off
      mask Display: e = 0.06;c1 = [120 230 180]/255;c2 = ([120 230 180]+0)/(256+128);c3 = ([120 230 180]+128)/(256+128);patch([0 1 1 0],[0 0 1 1],c1);patch([0 1 1 1-e 1-e 0+e],[0 0 1 1-e 0+e 0+e],c2);patch([0 0 1 1-e 0+e 0+e],[0 1 1 1-e 1-e 0+e],c3);plot([0 1 1 0 0],[0 0 1 1 0]);
  wires:
  "IW{2,1}(1,:)'"/1 -> dotprod1/1
  "ad{2,1}"/1 -> dotprod1/2
  dotprod1/1 -> Mux/1
  Mux/1 -> "lz{2,1}"/1
